simulink model "single_phase_ttype_inverter"  (R2026a)
settings: Solver=ode23tb  StopTime=simlength  FixedStep=tc  MaxStep=glb_time.tc
values from neighbouring files (symbols this model uses):
  afe_ctrl = param.afe.ctrl    [init_model.m]
  afe_pwm_phase_shift_mod1 = param.afe.behav.pwm_phase_shift_mod1    [init_model.m]
  DThs_init = param.thermal.DThs_init    [init_model.m]
  filters = param.ctrl.filters    [init_model.m]
  frt_data = param.frt.data    [init_model.m]
  glb_time = param.glb_time    [init_model.m]
  grid_emu = param.grid.emu    [init_model.m]
  kepsilon = param.spinv.kepsilon    [init_model.m]
  kp_align = param.ctrl.kp_align    [init_model.m]
  lim_down_align = param.ctrl.lim_down_align    [init_model.m]
  lim_up_align = param.ctrl.lim_up_align    [init_model.m]
  mavarage_filter_frequency_base_order = param.ctrl.mavarage_filter_frequency_base_order    [init_model.m]
  omega_set = param.spinv.omega_set    [init_model.m]
  single_phase_inverter_ctrl = param.spinv.ctrl    [init_model.m]
  Tambient = param.thermal.Tambient    [init_model.m]
  time_aux_power_supply_fault = param.sim.time_aux_power_supply_fault    [init_model.m]
  time_step_ref_1 = param.spinv.ref.time_step_ref_1    [init_model.m]
  time_step_ref_2 = param.spinv.ref.time_step_ref_2    [init_model.m]
  time_step_ref_3 = param.spinv.ref.time_step_ref_3    [init_model.m]
undefined symbols (not defined in the file or in its folder): delta_fht1, hwdata, ki_align, Ld_fht1, magnitude, omega_fht1, ts_inv, Vac_FS, Vdc_nom, Xbez
libraries: fl_lib x61, nesl_utility x39, moving_average_filter x11, moving_average_filter_cc x8, discrete_time_low_pass_filter x4, sl_discontinuities x3, single_phase_transformer_lib x3, linear_double_integrator_observer_ccaller x2, phase_shift_filter_ccaller x2, threephase_inductor_lib x1, dclink_for_two_levels x1, three_phase_pwm_modulator x1
(part 6 of 9)

== system single_phase_ttype_inverter/afe/AFE_control/afe_control/grid_voltage_phase_lock_loops/dq_pll_ccaller/first_harmonic_tracker_phase_u ==
  u : Inport
  Bus Selector : BusSelector  OutputSignals=output_pu_hat
  C Caller : CCaller  FunctionName=first_harmonic_tracker_process_simulink  PortSpecificationStruct="%)30     .    B \\   8    (     @         %    \"     D    !     0         %  0 \"0    $    _    07)G3F%M90  4&]R=$YA;64 4V-O<&4     26YD97@     5'EP90      4VEZ90      27-';&]B86P   X    P    !@    @    $          4    (     0    ,    !         !   P!O=70 #@   #     &    \"     0         !0    @    !     P    $         $  # &]U=  .    .     8    (    !          %    \"     $    &     0         0  ...(+4988 chars)"
  Constant : Constant  Value=glb_time.ts_afe
  Constant1 : Constant  Value=0
  Constant4 : Constant  Value=afe_ctrl.fht_grid.omega_fht
  Constant5 : Constant  Value=afe_ctrl.fht_grid.delta_fht
  Constant6 : Constant  Value=afe_ctrl.fht_grid.Ld_fht(1)
  Constant7 : Constant  Value=afe_ctrl.fht_grid.Ld_fht(2)
  Data Type Conversion{1..2,6..9} (6 alike) : DataTypeConversion  OutDataTypeStr=single  SaturateOnIntegerOverflow=off  RndMeth=Floor
  Data Type Conversion3 : DataTypeConversion  OutDataTypeStr=uint8  SaturateOnIntegerOverflow=off  RndMeth=Floor
  Data Type Conversion4 : DataTypeConversion  OutDataTypeStr=double  SaturateOnIntegerOverflow=off  RndMeth=Floor
  Data Type Conversion5 : DataTypeConversion  OutDataTypeStr=uint8  SaturateOnIntegerOverflow=off  RndMeth=Floor
  Step : Step  Time=0.0125  InitialValue=1  FinalValue=0
  u_hat : Outport
  wires:
  Data Type Conversion4/1 -> u_hat/1
  Data Type Conversion3/1 -> C Caller/1
  Data Type Conversion1/1 -> C Caller/3
  Data Type Conversion2/1 -> C Caller/2
  C Caller/1 -> Bus Selector/1
  Bus Selector/1 -> Data Type Conversion4/1  "<output_pu_hat>"
  Step/1 -> Data Type Conversion3/1
  u/1 -> Data Type Conversion2/1
  Constant/1 -> Data Type Conversion1/1
  Constant1/1 -> Data Type Conversion5/1
  Constant4/1 -> Data Type Conversion6/1
  Constant6/1 -> Data Type Conversion8/1
  Constant7/1 -> Data Type Conversion9/1
  Constant5/1 -> Data Type Conversion7/1
  Data Type Conversion5/1 -> C Caller/8
  Data Type Conversion6/1 -> C Caller/4
  Data Type Conversion7/1 -> C Caller/5
  Data Type Conversion8/1 -> C Caller/6
  Data Type Conversion9/1 -> C Caller/7

== system single_phase_ttype_inverter/afe/AFE_control/afe_control/grid_voltage_phase_lock_loops/dq_pll_ccaller/first_harmonic_tracker_phase_v ==
  u : Inport
  Bus Selector : BusSelector  OutputSignals=output_pu_hat
  C Caller : CCaller  FunctionName=first_harmonic_tracker_process_simulink  PortSpecificationStruct="%)30     .    B \\   8    (     @         %    \"     D    !     0         %  0 \"0    $    _    07)G3F%M90  4&]R=$YA;64 4V-O<&4     26YD97@     5'EP90      4VEZ90      27-';&]B86P   X    P    !@    @    $          4    (     0    ,    !         !   P!O=70 #@   #     &    \"     0         !0    @    !     P    $         $  # &]U=  .    .     8    (    !          %    \"     $    &     0         0  ...(+4988 chars)"
  Constant : Constant  Value=glb_time.ts_afe
  Constant1 : Constant  Value=2
  Constant4 : Constant  Value=afe_ctrl.fht_grid.omega_fht
  Constant5 : Constant  Value=afe_ctrl.fht_grid.delta_fht
  Constant6 : Constant  Value=afe_ctrl.fht_grid.Ld_fht(1)
  Constant7 : Constant  Value=afe_ctrl.fht_grid.Ld_fht(2)
  Data Type Conversion{1..2,6..9} (6 alike) : DataTypeConversion  OutDataTypeStr=single  SaturateOnIntegerOverflow=off  RndMeth=Floor
  Data Type Conversion3 : DataTypeConversion  OutDataTypeStr=uint8  SaturateOnIntegerOverflow=off  RndMeth=Floor
  Data Type Conversion4 : DataTypeConversion  OutDataTypeStr=double  SaturateOnIntegerOverflow=off  RndMeth=Floor
  Data Type Conversion5 : DataTypeConversion  OutDataTypeStr=uint8  SaturateOnIntegerOverflow=off  RndMeth=Floor
  Step : Step  Time=0.0125  InitialValue=1  FinalValue=0
  u_hat : Outport
  wires:
  Data Type Conversion9/1 -> C Caller/7
  Data Type Conversion8/1 -> C Caller/6
  Data Type Conversion7/1 -> C Caller/5
  Data Type Conversion6/1 -> C Caller/4
  Data Type Conversion5/1 -> C Caller/8
  Constant5/1 -> Data Type Conversion7/1
  Constant7/1 -> Data Type Conversion9/1
  Constant6/1 -> Data Type Conversion8/1
  Constant4/1 -> Data Type Conversion6/1
  Constant1/1 -> Data Type Conversion5/1
  Constant/1 -> Data Type Conversion1/1
  u/1 -> Data Type Conversion2/1
  Step/1 -> Data Type Conversion3/1
  Bus Selector/1 -> Data Type Conversion4/1  "<output_pu_hat>"
  C Caller/1 -> Bus Selector/1
  Data Type Conversion2/1 -> C Caller/2
  Data Type Conversion1/1 -> C Caller/3
  Data Type Conversion3/1 -> C Caller/1
  Data Type Conversion4/1 -> u_hat/1

== system single_phase_ttype_inverter/afe/AFE_control/afe_control/grid_voltage_phase_lock_loops/dq_pll_ccaller/first_harmonic_tracker_phase_w ==
  u : Inport
  Bus Selector : BusSelector  OutputSignals=output_pu_hat
  C Caller : CCaller  FunctionName=first_harmonic_tracker_process_simulink  PortSpecificationStruct="%)30     .    B \\   8    (     @         %    \"     D    !     0         %  0 \"0    $    _    07)G3F%M90  4&]R=$YA;64 4V-O<&4     26YD97@     5'EP90      4VEZ90      27-';&]B86P   X    P    !@    @    $          4    (     0    ,    !         !   P!O=70 #@   #     &    \"     0         !0    @    !     P    $         $  # &]U=  .    .     8    (    !          %    \"     $    &     0         0  ...(+4988 chars)"
  Constant : Constant  Value=glb_time.ts_afe
  Constant1 : Constant  Value=4
  Constant4 : Constant  Value=afe_ctrl.fht_grid.omega_fht
  Constant5 : Constant  Value=afe_ctrl.fht_grid.delta_fht
  Constant6 : Constant  Value=afe_ctrl.fht_grid.Ld_fht(1)
  Constant7 : Constant  Value=afe_ctrl.fht_grid.Ld_fht(2)
  Data Type Conversion{1..2,6..9} (6 alike) : DataTypeConversion  OutDataTypeStr=single  SaturateOnIntegerOverflow=off  RndMeth=Floor
  Data Type Conversion3 : DataTypeConversion  OutDataTypeStr=uint8  SaturateOnIntegerOverflow=off  RndMeth=Floor
  Data Type Conversion4 : DataTypeConversion  OutDataTypeStr=double  SaturateOnIntegerOverflow=off  RndMeth=Floor
  Data Type Conversion5 : DataTypeConversion  OutDataTypeStr=uint8  SaturateOnIntegerOverflow=off  RndMeth=Floor
  Step : Step  Time=0.0125  InitialValue=1  FinalValue=0
  u_hat : Outport
  wires:
  Data Type Conversion4/1 -> u_hat/1
  Data Type Conversion3/1 -> C Caller/1
  Data Type Conversion1/1 -> C Caller/3
  Data Type Conversion2/1 -> C Caller/2
  C Caller/1 -> Bus Selector/1
  Bus Selector/1 -> Data Type Conversion4/1  "<output_pu_hat>"
  Step/1 -> Data Type Conversion3/1
  u/1 -> Data Type Conversion2/1
  Constant/1 -> Data Type Conversion1/1
  Constant1/1 -> Data Type Conversion5/1
  Constant4/1 -> Data Type Conversion6/1
  Constant6/1 -> Data Type Conversion8/1
  Constant7/1 -> Data Type Conversion9/1
  Constant5/1 -> Data Type Conversion7/1
  Data Type Conversion5/1 -> C Caller/8
  Data Type Conversion6/1 -> C Caller/4
  Data Type Conversion7/1 -> C Caller/5
  Data Type Conversion8/1 -> C Caller/6
  Data Type Conversion9/1 -> C Caller/7

== system single_phase_ttype_inverter/afe/AFE_control/afe_control/grid_voltage_sequences/voltage_sequence_avg/average_filter ==
  v_grid_pos_xi : Inport
  v_grid_pos_eta : Inport  Port=2
  v_grid_neg_xi : Inport  Port=3
  v_grid_neg_eta : Inport  Port=4
  Abs : Abs  SaturateOnIntegerOverflow=off
  Gain : Gain  Gain=grid_emu.omega_grid_nom*mavarage_filter_frequency_base_order
  Saturation : Saturate  UpperLimit=2  LowerLimit=0.1
  dmavg_flt{,1..3} (4 alike) : moving_average_filter/dmavg_flt  ts=glb_time.ts_afe  enable_time=dmavg_filter_enable_time
  v_grid_pos_xi_avg : Outport
  v_grid_pos_eta_avg : Outport  Port=2
  v_grid_neg_xi_avg : Outport  Port=3
  v_grid_neg_eta_avg : Outport  Port=4
  wires:
  v_grid_neg_eta/1 -> dmavg_flt3/1
  v_grid_neg_xi/1 -> dmavg_flt2/1
  v_grid_pos_eta/1 -> dmavg_flt1/1
  dmavg_flt3/1 -> v_grid_neg_eta_avg/1
  dmavg_flt2/1 -> v_grid_neg_xi_avg/1
  dmavg_flt1/1 -> v_grid_pos_eta_avg/1
  Gain/1 -> dmavg_flt/2, dmavg_flt1/2, dmavg_flt2/2, dmavg_flt3/2
  dmavg_flt/1 -> v_grid_pos_xi_avg/1
  v_grid_pos_xi/1 -> dmavg_flt/1
  Abs/1 -> Saturation/1
  [omega_grid_pll_pu_mod1] -> Abs/1
  Saturation/1 -> Gain/1

== system single_phase_ttype_inverter/afe/AFE_control/afe_control/grid_voltage_sequences/voltage_sequence_avg/average_filter_ccaller ==
  v_grid_pos_xi : Inport
  v_grid_pos_eta : Inport  Port=2
  v_grid_neg_xi : Inport  Port=3
  v_grid_neg_eta : Inport  Port=4
  Abs : Abs  SaturateOnIntegerOverflow=off
  Gain : Gain  Gain=grid_emu.omega_grid_nom*mavarage_filter_frequency_base_order
  Saturation : Saturate  UpperLimit=2  LowerLimit=0.1
  dmavg_flt : moving_average_filter_cc/dmavg_flt  instance=0  ts=glb_time.ts_afe  enable_time=dmavg_filter_enable_time
  dmavg_flt1 : moving_average_filter_cc/dmavg_flt  instance=1  ts=glb_time.ts_afe  enable_time=dmavg_filter_enable_time
  dmavg_flt2 : moving_average_filter_cc/dmavg_flt  instance=2  ts=glb_time.ts_afe  enable_time=dmavg_filter_enable_time
  dmavg_flt3 : moving_average_filter_cc/dmavg_flt  instance=3  ts=glb_time.ts_afe  enable_time=dmavg_filter_enable_time
  v_grid_pos_xi_avg : Outport
  v_grid_pos_eta_avg : Outport  Port=2
  v_grid_neg_xi_avg : Outport  Port=3
  v_grid_neg_eta_avg : Outport  Port=4
  wires:
  v_grid_pos_xi/1 -> dmavg_flt/1
  dmavg_flt/1 -> v_grid_pos_xi_avg/1
  dmavg_flt1/1 -> v_grid_pos_eta_avg/1
  dmavg_flt2/1 -> v_grid_neg_xi_avg/1
  dmavg_flt3/1 -> v_grid_neg_eta_avg/1
  v_grid_pos_eta/1 -> dmavg_flt1/1
  v_grid_neg_xi/1 -> dmavg_flt2/1
  v_grid_neg_eta/1 -> dmavg_flt3/1
  Abs/1 -> Saturation/1
  Saturation/1 -> Gain/1
  [omega_grid_pll_pu_mod1] -> Abs/1
  Gain/1 -> dmavg_flt/2, dmavg_flt1/2, dmavg_flt3/2, dmavg_flt2/2

== system single_phase_ttype_inverter/afe/AFE_control/afe_control/phase_compensation_1/alignment_eval_afe1/pi ==
  u_ref : Inport
  u : Inport  Port=2
  1/Ti : Gain  Gain=kp  SaturateOnIntegerOverflow=on  OutDataTypeStr=Inherit: Same as input  ParamDataTypeStr=Inherit: Same as input
  Saturation : Saturate  UpperLimit=lim_up  LowerLimit=lim_down
  Sum1 : Sum  Inputs=+++  SaturateOnIntegerOverflow=on
  Sum2 : Sum  Inputs=-+  SaturateOnIntegerOverflow=on
  Sum3 : Sum  Inputs=-+  SaturateOnIntegerOverflow=on
  Unit Delay4 : UnitDelay  SampleTime=-1
  kp : Gain  Gain=ki  SaturateOnIntegerOverflow=on  OutDataTypeStr=Inherit: Same as input  ParamDataTypeStr=Inherit: Same as input
  y : Outport
  wires:
  1/Ti/1 -> Sum1/1, Sum3/1
  kp/1 -> Sum1/2
  Sum3/1 -> Unit Delay4/1
  Unit Delay4/1 -> Sum1/3
  u_ref/1 -> Sum2/2
  u/1 -> Sum2/1
  Sum2/1 -> kp/1, 1/Ti/1
  Sum1/1 -> Saturation/1
  Saturation/1 -> Sum3/2, y/1

== system single_phase_ttype_inverter/single_phase_inverter/single phase inverter control/single_phase_inverter_ctrl/phase generator/dq_pll_ccaller/dqpll_grid_ccaller ==
  reset : Inport
  phase_u : Inport  Port=2
  phase_v : Inport  Port=3
  phase_w : Inport  Port=4
  ts : Inport  Port=5
  Bus Selector : BusSelector  OutputSignals=omega_pu_hat,gamma_hat,u_grid_xi,u_grid_eta,dqpll_pll_state
  Data Type Conversion{1..2,4..5} (4 alike) : DataTypeConversion  OutDataTypeStr=single  SaturateOnIntegerOverflow=off  RndMeth=Floor
  Data Type Conversion{6..10} (5 alike) : DataTypeConversion  OutDataTypeStr=double  SaturateOnIntegerOverflow=off  RndMeth=Floor
  Data Type Conversion3 : DataTypeConversion  OutDataTypeStr=uint8  SaturateOnIntegerOverflow=off  RndMeth=Floor
  Zero-Order Hold{,1..4} (5 alike) : ZeroOrderHold  SampleTime=-1
  dqpll_grid : CCaller  FunctionName=dqpll_grid_process_simulink  PortSpecificationStruct="%)30     .    N H   8    (     @         %    \"     8    !     0         %  0 \"0    $    _    07)G3F%M90  4&]R=$YA;64 4V-O<&4     26YD97@     5'EP90      4VEZ90      27-';&]B86P   X    P    !@    @    $          4    (     0    ,    !         !   P!O=70 #@   #     &    \"     0         !0    @    !     P    $         $  # &]U=  .    .     8    (    !          %    \"     $    &     0         0   ...(+3319 chars)"
  gamma_hat : Outport  VectorParamsAs1DForOutWhenUnconnected=off
  omega_pu_hat : Outport  Port=2  VectorParamsAs1DForOutWhenUnconnected=off
  dqpll_uxi : Outport  Port=3  VectorParamsAs1DForOutWhenUnconnected=off
  dqpll_ueta : Outport  Port=4  VectorParamsAs1DForOutWhenUnconnected=off
  dqpll_state : Outport  Port=5  VectorParamsAs1DForOutWhenUnconnected=off
  wires:
  Bus Selector/1 -> Data Type Conversion6/1  "<omega_pu_hat>"
  Data Type Conversion7/1 -> gamma_hat/1
  Bus Selector/2 -> Data Type Conversion7/1  "<gamma_hat>"
  dqpll_grid/1 -> Bus Selector/1
  phase_v/1 -> Zero-Order Hold2/1
  Bus Selector/3 -> Data Type Conversion8/1  "<u_grid_xi>"
  Data Type Conversion5/1 -> dqpll_grid/4
  Bus Selector/4 -> Data Type Conversion9/1  "<u_grid_eta>"
  reset/1 -> Zero-Order Hold/1
  Data Type Conversion10/1 -> dqpll_state/1
  Bus Selector/5 -> Data Type Conversion10/1  "<dqpll_pll_state>"
  Data Type Conversion4/1 -> dqpll_grid/3
  Data Type Conversion1/1 -> dqpll_grid/5
  phase_u/1 -> Zero-Order Hold1/1
  Data Type Conversion3/1 -> dqpll_grid/1
  phase_w/1 -> Zero-Order Hold3/1
  Data Type Conversion2/1 -> dqpll_grid/2
  Data Type Conversion9/1 -> dqpll_ueta/1
  Data Type Conversion6/1 -> omega_pu_hat/1
  Data Type Conversion8/1 -> dqpll_uxi/1
  ts/1 -> Zero-Order Hold4/1
  Zero-Order Hold/1 -> Data Type Conversion3/1
  Zero-Order Hold1/1 -> Data Type Conversion2/1
  Zero-Order Hold2/1 -> Data Type Conversion4/1
  Zero-Order Hold3/1 -> Data Type Conversion5/1
  Zero-Order Hold4/1 -> Data Type Conversion1/1

== system single_phase_ttype_inverter/single_phase_inverter/single phase inverter control/single_phase_inverter_ctrl/phase generator/dq_pll_ccaller/first_harmonic_tracker1 ==
  u : Inport
  Bus Selector : BusSelector  OutputSignals=output_pu_hat
  Constant : Constant  Value=glb_time.ts_inv
  Constant1 : Constant  Value=0
  Constant2 : Constant  Value=afe_ctrl.fht_grid.omega_fht
  Constant3 : Constant  Value=afe_ctrl.fht_grid.delta_fht
  Constant4 : Constant  Value=afe_ctrl.fht_grid.Ld_fht(1)
  Constant5 : Constant  Value=afe_ctrl.fht_grid.Ld_fht(2)
  Data Type Conversion{1..2,6..9} (6 alike) : DataTypeConversion  OutDataTypeStr=single  SaturateOnIntegerOverflow=off  RndMeth=Floor
  Data Type Conversion3 : DataTypeConversion  OutDataTypeStr=uint8  SaturateOnIntegerOverflow=off  RndMeth=Floor
  Data Type Conversion4 : DataTypeConversion  OutDataTypeStr=double  SaturateOnIntegerOverflow=off  RndMeth=Floor
  Data Type Conversion5 : DataTypeConversion  OutDataTypeStr=uint8  SaturateOnIntegerOverflow=off  RndMeth=Floor
  Step : Step  Time=0.0125  InitialValue=1  FinalValue=0
  first_harmonic_tracker : CCaller  FunctionName=first_harmonic_tracker_process_simulink  PortSpecificationStruct="%)30     .    B \\   8    (     @         %    \"     D    !     0         %  0 \"0    $    _    07)G3F%M90  4&]R=$YA;64 4V-O<&4     26YD97@     5'EP90      4VEZ90      27-';&]B86P   X    P    !@    @    $          4    (     0    ,    !         !   P!O=70 #@   #     &    \"     0         !0    @    !     P    $         $  # &]U=  .    .     8    (    !          %    \"     $    &     0         0  ...(+4988 chars)"
  u_hat : Outport
  wires:
  Data Type Conversion4/1 -> u_hat/1
  Data Type Conversion3/1 -> first_harmonic_tracker/1
  Data Type Conversion1/1 -> first_harmonic_tracker/3
  Data Type Conversion2/1 -> first_harmonic_tracker/2
  first_harmonic_tracker/1 -> Bus Selector/1
  Bus Selector/1 -> Data Type Conversion4/1  "<output_pu_hat>"
  Step/1 -> Data Type Conversion3/1
  u/1 -> Data Type Conversion2/1
  Constant/1 -> Data Type Conversion1/1
  Constant1/1 -> Data Type Conversion5/1
  Data Type Conversion5/1 -> first_harmonic_tracker/8
  Constant2/1 -> Data Type Conversion6/1
  Data Type Conversion6/1 -> first_harmonic_tracker/4
  Constant3/1 -> Data Type Conversion7/1
  Data Type Conversion7/1 -> first_harmonic_tracker/5
  Constant4/1 -> Data Type Conversion8/1
  Data Type Conversion8/1 -> first_harmonic_tracker/6
  Constant5/1 -> Data Type Conversion9/1
  Data Type Conversion9/1 -> first_harmonic_tracker/7

== system single_phase_ttype_inverter/single_phase_inverter/single phase inverter control/single_phase_inverter_ctrl/phase generator/dq_pll_ccaller/first_harmonic_tracker2 ==
  u : Inport
  Bus Selector : BusSelector  OutputSignals=output_pu_hat
  Constant : Constant  Value=glb_time.ts_inv
  Constant1 : Constant  Value=2
  Constant2 : Constant  Value=afe_ctrl.fht_grid.omega_fht
  Constant3 : Constant  Value=afe_ctrl.fht_grid.delta_fht
  Constant4 : Constant  Value=afe_ctrl.fht_grid.Ld_fht(1)
  Constant5 : Constant  Value=afe_ctrl.fht_grid.Ld_fht(2)
  Data Type Conversion{1..2,6..9} (6 alike) : DataTypeConversion  OutDataTypeStr=single  SaturateOnIntegerOverflow=off  RndMeth=Floor
  Data Type Conversion3 : DataTypeConversion  OutDataTypeStr=uint8  SaturateOnIntegerOverflow=off  RndMeth=Floor
  Data Type Conversion4 : DataTypeConversion  OutDataTypeStr=double  SaturateOnIntegerOverflow=off  RndMeth=Floor
  Data Type Conversion5 : DataTypeConversion  OutDataTypeStr=uint8  SaturateOnIntegerOverflow=off  RndMeth=Floor
  Step : Step  Time=0.0125  InitialValue=1  FinalValue=0
  first_harmonic_tracker : CCaller  FunctionName=first_harmonic_tracker_process_simulink  PortSpecificationStruct="%)30     .    B \\   8    (     @         %    \"     D    !     0         %  0 \"0    $    _    07)G3F%M90  4&]R=$YA;64 4V-O<&4     26YD97@     5'EP90      4VEZ90      27-';&]B86P   X    P    !@    @    $          4    (     0    ,    !         !   P!O=70 #@   #     &    \"     0         !0    @    !     P    $         $  # &]U=  .    .     8    (    !          %    \"     $    &     0         0  ...(+4988 chars)"
  u_hat : Outport
  wires:
  Data Type Conversion9/1 -> first_harmonic_tracker/7
  Constant5/1 -> Data Type Conversion9/1
  Data Type Conversion8/1 -> first_harmonic_tracker/6
  Constant4/1 -> Data Type Conversion8/1
  Data Type Conversion7/1 -> first_harmonic_tracker/5
  Constant3/1 -> Data Type Conversion7/1
  Data Type Conversion6/1 -> first_harmonic_tracker/4
  Constant2/1 -> Data Type Conversion6/1
  Data Type Conversion5/1 -> first_harmonic_tracker/8
  Constant1/1 -> Data Type Conversion5/1
  Constant/1 -> Data Type Conversion1/1
  u/1 -> Data Type Conversion2/1
  Step/1 -> Data Type Conversion3/1
  Bus Selector/1 -> Data Type Conversion4/1  "<output_pu_hat>"
  first_harmonic_tracker/1 -> Bus Selector/1
  Data Type Conversion2/1 -> first_harmonic_tracker/2
  Data Type Conversion1/1 -> first_harmonic_tracker/3
  Data Type Conversion3/1 -> first_harmonic_tracker/1
  Data Type Conversion4/1 -> u_hat/1
